simulink model "enlace_fibra_8QAM"  (R2026b)
settings: Solver=FixedStepDiscrete  StopTime=inf
InitFcn:
  | init_params
values from neighbouring files (symbols this model uses):
  delayBits = k*delaySym + delayErr    [init_derived.m]
  hCD = delta;  if useCD,     hCD     = fftshift(ifft(ifftshift(H)));       end    [init_derived.m]
  hCDcomp = delta;  if useCDcomp, hCDcomp = fftshift(ifft(ifftshift(conj(H)))); end    [init_derived.m]
  K = sqrt(Ga)    [init_derived.m]
  Kin = sqrt(P0)    [init_derived.m]
  Krx = 1/(K*Kin)    [init_derived.m]
  Ts = 1/Rs    [init_derived.m]
undefined symbols (not defined in the file or in its folder): rolloff, sps
libraries: commfilt2 x3, commdigbbndam3 x2, simulink x2, commchan3 x1, commsink2 x1, commrandsrc3 x1
settings Model: Creator=matiasjesusdiazllancan  LastModifiedBy=matiasjesusdiazllancan

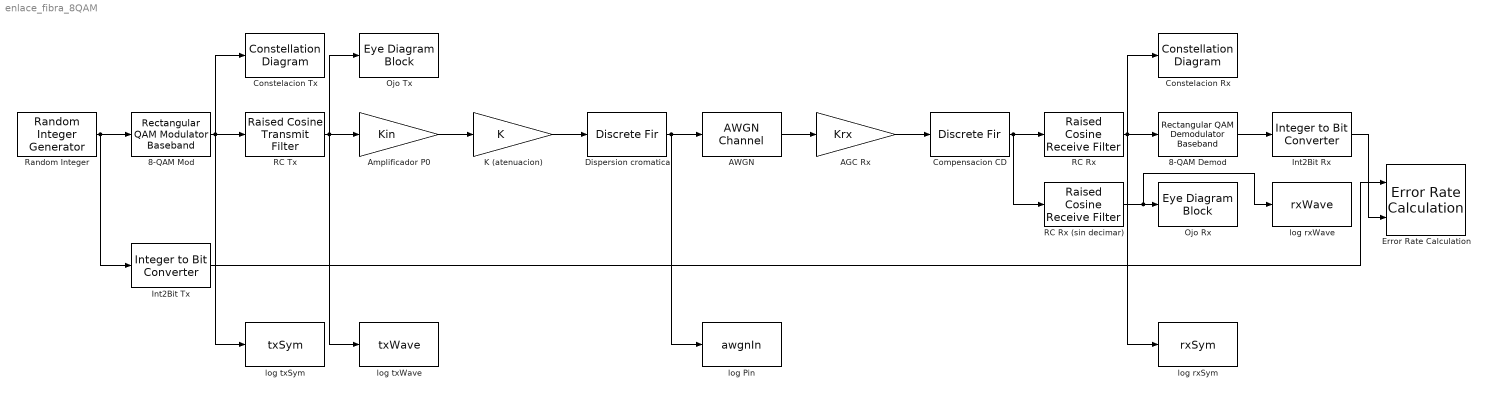
== system enlace_fibra_8QAM ==
  8-QAM Demod : commdigbbndam3/Rectangular QAM Demodulator Baseband  M=M  OutType=Integer  DecType=Hard decision  VarSource=Dialog  Variance=1  Dec=Gray  Mapping=[0:15]  PowType=Average Power  MinDist=2  AvgPow=1  PeakPow=1  Ph=0  outDtype1=Inherit via internal rule  outDtype2=Inherit via internal rule  derotateFactorWordLen=16  derotateFactorDataTypeStr=Inherit: Same word length as input  derotateFactorLastDataTypeStr=Inherit: Same word length as input  denormFactorWordLen=16  denormFactorDataTypeStr=Inherit: Same word length as input  denormFactorLastDataTypeStr=Inherit: Same word length as input  prodOutWordLen=32  prodOutOverflowMode=Wrap  prodOutRoundingMode=Floor  prodOutOvFlMode=off  prodOutOvFlModeLastStrValue=off  sumWordLen=32
  8-QAM Mod : commdigbbndam3/Rectangular QAM Modulator Baseband  M=M  InType=Integer  Enc=Gray  Mapping=[0:15]  PowType=Average Power  MinDist=2  AvgPow=1  PeakPow=1  Ph=0  outDtype=double  outWordLen=16  outUDDataType=sfix(16)  outFracLenMode=Best precision  outFracLen=15  outDataTypeStr=double  outLastDataTypeStr=double
  AGC Rx : Gain  Gain=Krx
  AWGN : commchan3/AWGN Channel  LegacyMode=off  NoiseMethod="Signal to noise ratio  (Eb/No)"  noiseMode="Signal to noise ratio  (Eb/No)"  EbNo=EbNo  EsNo=10  SNR=10  BitsPerSymbol=k  SignalPower=Psig  SpecifySymbolPeriod=off  SamplesPerSymbol=sps  SymbolPeriod=1  VarianceSource=Parameter  Variance=1  RandomStream=Global stream  Seed=67  SimulateUsing=Code generation
  Amplificador P0 : Gain  Gain=Kin
  Compensacion CD : DiscreteFir  Coefficients=hCDcomp  InputProcessing=Columns as channels (frame based)
  Constelacion Rx : ConstellationDiagram
  Constelacion Tx : ConstellationDiagram
  Dispersion cromatica : DiscreteFir  Coefficients=hCD  InputProcessing=Columns as channels (frame based)
  Error Rate Calculation : commsink2/Error Rate Calculation  N=delayBits  st_delay=0  cp_mode=Entire frame  subframe=[]  PMode=Workspace  WsName=BER  RsMode2=off  stop=on  numErr=maxNumErrs  maxBits=maxNumBits
  Int2Bit Rx : simulink/Logic and Bit Operations/Integer to Bit Converter  nbits=k  signedInputValues=Unsigned  bitOrder=MSB first  outDtype=Inherit via internal rule
      settings: LibrarySourceBlock=|
      | commutil2/Integer to Bit
      | Converter
  Int2Bit Tx : simulink/Logic and Bit Operations/Integer to Bit Converter  nbits=k  signedInputValues=Unsigned  bitOrder=MSB first  outDtype=Inherit via internal rule
      settings: LibrarySourceBlock=|
      | commutil2/Integer to Bit
      | Converter
  K (atenuacion) : Gain  Gain=K
  Ojo Rx : EyeDiagramBlock  SamplesPerSymbol=sps
  Ojo Tx : EyeDiagramBlock  SamplesPerSymbol=sps
  RC Rx : commfilt2/Raised Cosine Receive Filter  filtType=Square root  R=rolloff  filtSpan=span  N=sps  downFactor=sps  downOffset=0  filterGain=1  InputProcessing=Columns as channels (frame based)  RateOptions=Enforce single-rate processing  framing=Mute  checkCoeff=off  variableName=rcRxFilt  currentFiltSpan=10  D=5  inputOffset=0  sampMode=Mute  saveAsFlag=0  rateMode=Downsampling  checkGain=Normalized  launchFVT=on  roundingMode=Floor  overflowMode=off  coeffDataTypeStr=Inherit: Same word length as input  coeffMin=[]  coeffMax=[]  coeffLastDataTypeStr=Inherit: Same word length as input  accumDataTypeStr=Inherit: Same as product output  accumLastDataTypeStr=Inherit: Same as product output  outputDataTypeStr=Inherit: Same as accumulator  outputMin=[]  outputMax=[]  outputLastDataTypeStr=Inherit: Same as accumulator
  RC Rx (sin decimar) : commfilt2/Raised Cosine Receive Filter  filtType=Square root  R=rolloff  filtSpan=span  N=sps  downFactor=1  downOffset=0  filterGain=1  InputProcessing=Columns as channels (frame based)  RateOptions=Enforce single-rate processing  framing=Mute  checkCoeff=off  variableName=rcRxFilt  currentFiltSpan=10  D=5  inputOffset=0  sampMode=Mute  saveAsFlag=0  rateMode=Downsampling  checkGain=Normalized  launchFVT=on  roundingMode=Floor  overflowMode=off  coeffDataTypeStr=Inherit: Same word length as input  coeffMin=[]  coeffMax=[]  coeffLastDataTypeStr=Inherit: Same word length as input  accumDataTypeStr=Inherit: Same as product output  accumLastDataTypeStr=Inherit: Same as product output  outputDataTypeStr=Inherit: Same as accumulator  outputMin=[]  outputMax=[]  outputLastDataTypeStr=Inherit: Same as accumulator
  RC Tx : commfilt2/Raised Cosine Transmit Filter  filtType=Square root  R=rolloff  filtSpan=span  N=sps  filterGain=1  InputProcessing=Columns as channels (frame based)  RateOptions=Enforce single-rate processing  framing=Mute  checkCoeff=off  variableName=rcTxFilt  checkGain=Normalized  sampMode=Mute  saveAsFlag=0  currentFiltSpan=10  D=(10)/2  launchFVT=on  roundingMode=Floor  overflowMode=off  coeffDataTypeStr=Inherit: Same word length as input  coeffMin=[]  coeffMax=[]  coeffLastDataTypeStr=Inherit: Same word length as input  outputDataTypeStr=Inherit: Same as accumulator  outputMin=[]  outputMax=[]  outputLastDataTypeStr=Inherit: Same as accumulator
  Random Integer : commrandsrc3/Random Integer Generator  SetSize=M  SeedSource=Auto  Seed=0  SampleTime=Ts  SamplesPerFrame=frameLen  OutputDataType=double  SimulateUsing=Interpreted execution
  log Pin : ToWorkspace  VariableName=awgnIn  SampleTime=-1
      settings: MaxDataPoints=logPts
  log rxSym : ToWorkspace  VariableName=rxSym  SampleTime=-1
      settings: MaxDataPoints=logPts
  log rxWave : ToWorkspace  VariableName=rxWave  SampleTime=-1
      settings: MaxDataPoints=logPts
  log txSym : ToWorkspace  VariableName=txSym  SampleTime=-1
      settings: MaxDataPoints=logPts
  log txWave : ToWorkspace  VariableName=txWave  SampleTime=-1
      settings: MaxDataPoints=logPts
  wires:
  Random Integer/1 -> 8-QAM Mod/1, Int2Bit Tx/1
  8-QAM Mod/1 -> RC Tx/1, Constelacion Tx/1, log txSym/1
  RC Tx/1 -> Amplificador P0/1, Ojo Tx/1, log txWave/1
  Amplificador P0/1 -> K (atenuacion)/1
  K (atenuacion)/1 -> Dispersion cromatica/1
  Dispersion cromatica/1 -> AWGN/1, log Pin/1
  AWGN/1 -> AGC Rx/1
  AGC Rx/1 -> Compensacion CD/1
  Compensacion CD/1 -> RC Rx/1, RC Rx (sin decimar)/1
  RC Rx/1 -> 8-QAM Demod/1, Constelacion Rx/1, log rxSym/1
  8-QAM Demod/1 -> Int2Bit Rx/1
  Int2Bit Rx/1 -> Error Rate Calculation/2
  Int2Bit Tx/1 -> Error Rate Calculation/1
  RC Rx (sin decimar)/1 -> Ojo Rx/1, log rxWave/1
